simulink model "LQR_linear_sim"  (R2026a)
settings: Solver=VariableStepAuto
undefined symbols (not defined in the file): A, B, C, K, L, Nr
settings Model: Creator=rebec  LastModifiedBy=rebec

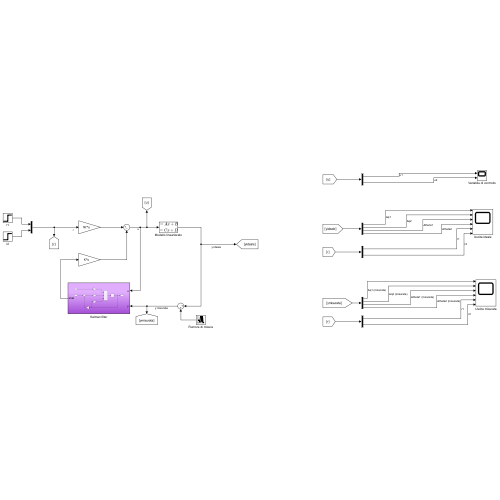
[thumbnail: Simulink's stored preview of the top-level diagram]
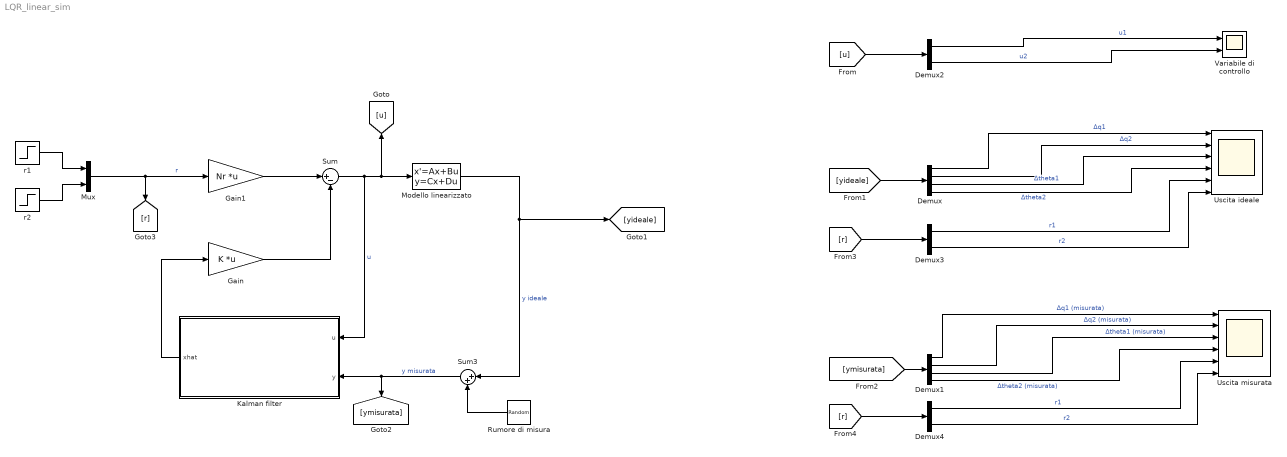
== system LQR_linear_sim ==
  Demux : Demux
  Demux1 : Demux
  Demux2 : Demux  Outputs=2
  Demux3 : Demux  Outputs=2
  Demux4 : Demux  Outputs=2
  Gain : Gain  Gain=K  Multiplication=Matrix(K*u)
  Gain1 : Gain  Gain=Nr  Multiplication=Matrix(K*u)
  Kalman filter : Subsystem
  Modello linearizzato : StateSpace  A=A  B=B  C=C  D=zeros(4,2);  InitialCondition=0
  Mux : Mux  Inputs=2
  Rumore di misura : RandomNumber  Variance=(0.05*pi/180)^2  Seed=20260826  SampleTime=0.002
  Sum : Sum  Inputs=|+-
  Sum3 : Sum  Inputs=|++
  Uscita ideale : Scope  NumInputPorts=6
      settings: Title=y (uscita ideale)  ActiveDisplayYMinimum=-0.12429032243772611  ActiveDisplayYMaximum=0.28578182686663178
  Uscita misurata : Scope  NumInputPorts=6
      settings: Title=y (uscita ideale)  ActiveDisplayYMinimum=-0.11442029066688837  ActiveDisplayYMaximum=0.16914890182413583
  Variabile di controllo : Scope  NumInputPorts=2
      settings: ActiveDisplayYMinimum=-2.6959450601265313  ActiveDisplayYMaximum=5.9059369724787079  DataLoggingVariableName=ScopeData2
  r1 : Step  FinalValue=5*pi/180  SampleTime=0
  r2 : Step  FinalValue=0  SampleTime=0
  wires:
  Demux/4 -> Uscita ideale/4  "Δtheta2"
  Demux2/1 -> Variabile di controllo/1  "u1"
  Demux1/1 -> Uscita misurata/1  "Δq1 (misurata)"
  r2/1 -> Mux/2
  Demux1/4 -> Uscita misurata/4  "Δtheta2 (misurata)"
  Rumore di misura/1 -> Sum3/2
  [r] -> Demux3/1
  Demux1/3 -> Uscita misurata/3  "Δtheta1 (misurata)"
  [u] -> Demux2/1
  [ymisurata] -> Demux1/1
  Demux3/1 -> Uscita ideale/5  "r1"
  Demux/1 -> Uscita ideale/1  "Δq1"
  Demux4/1 -> Uscita misurata/5  "r1"
  Demux1/2 -> Uscita misurata/2  "Δq2 (misurata)"
  Modello linearizzato/1 -> Sum3/1, [yideale]  "y ideale"
  Sum3/1 -> [ymisurata], Kalman filter/2(y)  "y misurata"
  r1/1 -> Mux/1
  Gain1/1 -> Sum/1
  [yideale] -> Demux/1
  Demux2/2 -> Variabile di controllo/2  "u2"
  Demux/2 -> Uscita ideale/2  "Δq2"
  Demux/3 -> Uscita ideale/3  "Δtheta1"
  Demux3/2 -> Uscita ideale/6  "r2"
  Sum/1 -> Modello linearizzato/1, [u], Kalman filter/1(u)  "u"
  Demux4/2 -> Uscita misurata/6  "r2"
  Mux/1 -> [r], Gain1/1  "r"
  [r] -> Demux4/1
  Kalman filter/1(xhat) -> Gain/1
  Gain/1 -> Sum/2

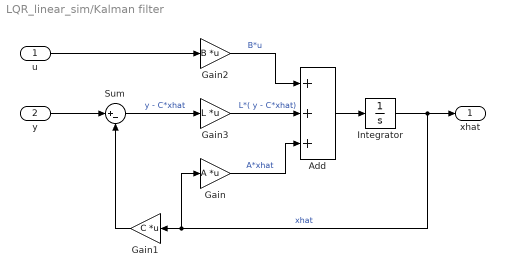
== system LQR_linear_sim/Kalman filter ==
  u : Inport
  y : Inport  Port=2
  Add : Sum  Inputs=+++
  Gain : Gain  Gain=A  Multiplication=Matrix(K*u)
  Gain1 : Gain  Gain=C  Multiplication=Matrix(K*u)
  Gain2 : Gain  Gain=B  Multiplication=Matrix(K*u)
  Gain3 : Gain  Gain=L  Multiplication=Matrix(K*u)
  Integrator : Integrator
  Sum : Sum  Inputs=|+-
  xhat : Outport
  wires:
  u/1 -> Gain2/1
  y/1 -> Sum/1
  Gain1/1 -> Sum/2
  Sum/1 -> Gain3/1  "y - C*xhat"
  Gain3/1 -> Add/2  "L*( y - C*xhat)"
  Gain2/1 -> Add/1  "B*u"
  Gain/1 -> Add/3  "A*xhat"
  Add/1 -> Integrator/1
  Integrator/1 -> Gain/1, Gain1/1, xhat/1  "xhat"
